simulink model "AirplaneSimModel"  (R2023b)
settings: Solver=ode45  StartTime=0.0  StopTime=inf  RelTol=1e-3
undefined symbols (not defined in the file): aileron_left, aileron_right, airplane, alt_ground, atmosphere, elevator, envir, g, htp_trim, rudder, throttle, wind
libraries: unit_conversions_lib x6, flightgear_visualization_lib x2, joystick_lib x1, conventional_airplane_single_engine_lib x1, atmosphere_lib x1, simulink x1
settings Model: Creator=Yannic  LastModifiedBy=yannic
settings SolverCC: AlgebraicLoopSolver=TrustRegion
settings DataIOCC: ReturnWorkspaceOutputs=off
settings DebuggingCC: UnconnectedInputMsg=warning  UnconnectedOutputMsg=warning  UnconnectedLineMsg=warning  ArithmeticOperatorsInVariantConditions=warning
settings ModelReferenceCC: EnableRefExpFcnMdlSchedulingChecks=on
settings SFSimCC: CustomCodeUndefinedFunction=UseInterfaceOnly

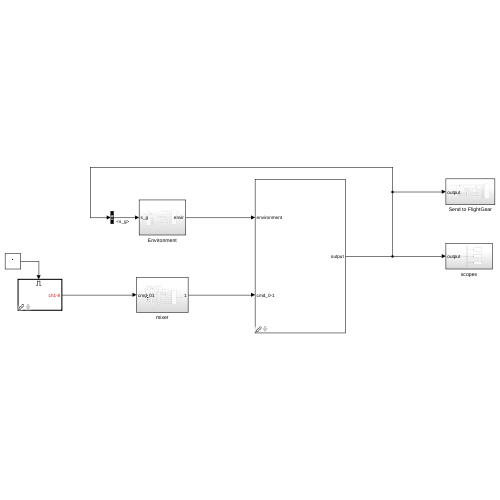
[thumbnail: Simulink's stored preview of the top-level diagram]
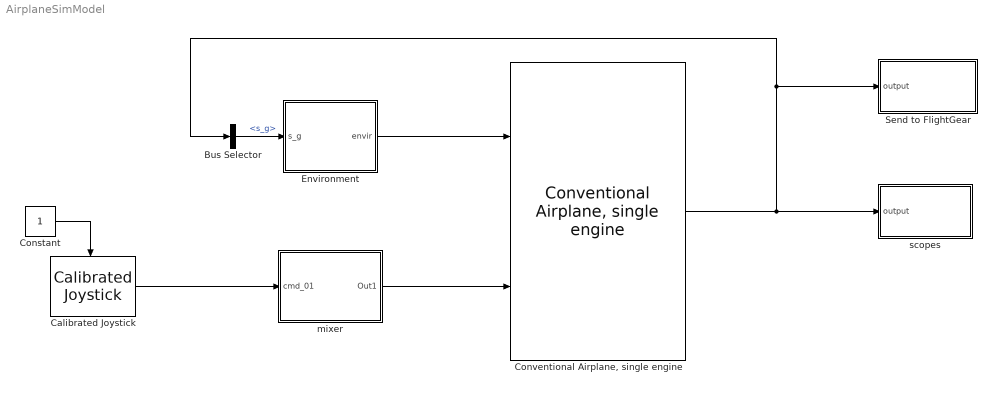
== system AirplaneSimModel ==
  Bus Selector : BusSelector  OutputSignals=rigidBodyBus.s_g
  Calibrated Joystick : joystick_lib/Calibrated Joystick  jystck=jystck  joyid=1
      settings: SourceProductName=LADAC
  Constant : Constant
  "Conventional Airplane, single engine" : conventional_airplane_single_engine_lib/Conventional Airplane, single engine  airplane=airplane
      settings: SourceProductName=LADAC
  Environment : Subsystem
  Send to FlightGear : Subsystem
  mixer : Subsystem
  scopes : Subsystem
  wires:
  Environment/1(envir) -> "Conventional Airplane, single engine"/1
  "Conventional Airplane, single engine"/1 -> Bus Selector/1, Send to FlightGear/1(output), scopes/1(output)
  mixer/1(Out1) -> "Conventional Airplane, single engine"/2
  Bus Selector/1 -> Environment/1(s_g)  "<s_g>"
  Constant/1 -> Calibrated Joystick/Enable
  Calibrated Joystick/1 -> mixer/1(cmd_01)

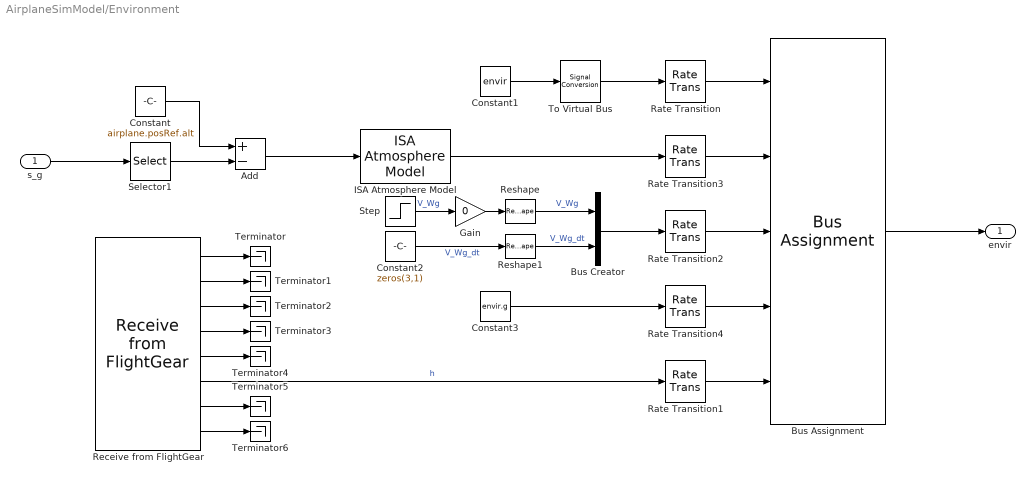
== system AirplaneSimModel/Environment ==
  s_g : Inport
  Add : Sum  Inputs=+-
  Bus Assignment : BusAssignment  AssignedSignals=atmosphere,wind,g,alt_ground
  Bus Creator : BusCreator  Inputs=2
  Constant : Constant  Value=airplane.posRef.alt
  Constant1 : Constant  Value=envir  OutDataTypeStr=Bus: envirBus
  Constant2 : Constant  Value=zeros(3,1)
  Constant3 : Constant  Value=envir.g
  Gain : Gain  Gain=0
  ISA Atmosphere Model : atmosphere_lib/ISA Atmosphere Model
      settings: SourceProductName=LADAC
  Rate Transition{,1..4} (5 alike) : RateTransition
  Receive from FlightGear : flightgear_visualization_lib/Receive from FlightGear  ip_address='127.0.0.1'  ip_port=5503  sample_time=1/40  blocking_time=0  is_aerocntrl=off  is_engine=off  is_fuel=off  is_land=off  is_avionics=off  is_envir=on
      settings: SourceProductName=LADAC
  Reshape : Reshape  OutputDimensionality=Column vector (2-D)
  Reshape1 : Reshape  OutputDimensionality=Column vector (2-D)
  Selector1 : Selector  InputPortWidth=3  IndexOptions=Index vector (dialog)  Indices=3  OutputSizes=1
  Step : Step  Time=3  After=[0;10;0]  SampleTime=0
  Terminator{,1..6} (7 alike) : Terminator
  To Virtual Bus : SignalConversion  ConversionOutput=Virtual bus  OverrideOpt=off
  envir : Outport  VectorParamsAs1DForOutWhenUnconnected=off
  wires:
  Receive from FlightGear/6 -> Rate Transition1/1  "h"
  Rate Transition2/1 -> Bus Assignment/3
  Rate Transition3/1 -> Bus Assignment/2
  Bus Assignment/1 -> envir/1
  Rate Transition/1 -> Bus Assignment/1
  ISA Atmosphere Model/1 -> Rate Transition3/1
  Step/1 -> Gain/1  "V_Wg"
  Rate Transition1/1 -> Bus Assignment/5
  Constant1/1 -> To Virtual Bus/1
  s_g/1 -> Selector1/1
  Bus Creator/1 -> Rate Transition2/1
  Constant2/1 -> Reshape1/1  "V_Wg_dt"
  Rate Transition4/1 -> Bus Assignment/4
  Constant3/1 -> Rate Transition4/1
  Gain/1 -> Reshape/1
  Constant/1 -> Add/1
  Add/1 -> ISA Atmosphere Model/1
  Selector1/1 -> Add/2
  To Virtual Bus/1 -> Rate Transition/1
  Reshape/1 -> Bus Creator/1  "V_Wg"
  Reshape1/1 -> Bus Creator/2  "V_Wg_dt"
  Receive from FlightGear/3 -> Terminator2/1
  Receive from FlightGear/5 -> Terminator4/1
  Receive from FlightGear/1 -> Terminator/1
  Receive from FlightGear/7 -> Terminator5/1
  Receive from FlightGear/2 -> Terminator1/1
  Receive from FlightGear/4 -> Terminator3/1
  Receive from FlightGear/8 -> Terminator6/1

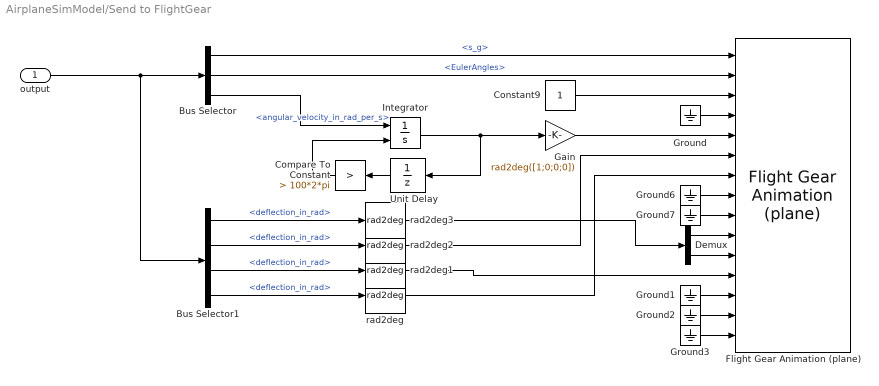
== system AirplaneSimModel/Send to FlightGear ==
  output : Inport
  Bus Selector : BusSelector  OutputSignals=rigidBodyBus.s_g,rigidBodyBus.EulerAngles,actuatorBus.motorBus.angular_velocity_in_rad_per_s
  Bus Selector1 : BusSelector  OutputSignals=actuatorBus.aileronsBus.deflection_in_rad,actuatorBus.elevatorBus.deflection_in_rad,actuatorBus.rudderBus.deflection_in_rad,actuatorBus.htpTrimBus.deflection_in_rad
  Compare To Constant : simulink/Logic and Bit Operations/Compare To Constant  relop=>  const=100*2*pi  OutDataTypeStr=boolean
  Constant9 : Constant
  Demux : Demux  Outputs=2
  Flight Gear Animation (plane) : flightgear_visualization_lib/Flight Gear Animation (plane)  inital_lat=airplane.posRef.lat  inital_long=airplane.posRef.lon  inital_height=airplane.posRef.alt  remoteURL='127.0.0.1'  remotePort=5502
      settings: SourceProductName=LADAC
  Gain : Gain  Gain=rad2deg([1;0;0;0])
  Ground{,1..3,6..7} (6 alike) : Ground
  Integrator : Integrator  ExternalReset=rising
  Unit Delay : UnitDelay  SampleTime=-1  HasFrameUpgradeWarning=on
  rad2deg{,1..3} (4 alike) : unit_conversions_lib/rad2deg
      settings: SourceProductName=LADAC
  wires:
  Compare To Constant/1 -> Integrator/2
  Integrator/1 -> Unit Delay/1, Gain/1
  Bus Selector/1 -> Flight Gear Animation (plane)/1  "<s_g>"
  Bus Selector/2 -> Flight Gear Animation (plane)/2  "<EulerAngles>"
  Gain/1 -> Flight Gear Animation (plane)/5
  Constant9/1 -> Flight Gear Animation (plane)/3
  Unit Delay/1 -> Compare To Constant/1
  Ground/1 -> Flight Gear Animation (plane)/4
  Ground1/1 -> Flight Gear Animation (plane)/13
  Ground2/1 -> Flight Gear Animation (plane)/14
  Ground3/1 -> Flight Gear Animation (plane)/15
  output/1 -> Bus Selector1/1, Bus Selector/1
  Bus Selector/3 -> Integrator/1  "<angular_velocity_in_rad_per_s>"
  Bus Selector1/2 -> rad2deg2/1  "<deflection_in_rad>"
  Bus Selector1/4 -> rad2deg/1  "<deflection_in_rad>"
  Ground6/1 -> Flight Gear Animation (plane)/8
  Ground7/1 -> Flight Gear Animation (plane)/9
  Bus Selector1/3 -> rad2deg1/1  "<deflection_in_rad>"
  Bus Selector1/1 -> rad2deg3/1  "<deflection_in_rad>"
  Demux/1 -> Flight Gear Animation (plane)/10
  Demux/2 -> Flight Gear Animation (plane)/11
  rad2deg/1 -> Flight Gear Animation (plane)/7
  rad2deg1/1 -> Flight Gear Animation (plane)/12
  rad2deg2/1 -> Flight Gear Animation (plane)/6
  rad2deg3/1 -> Demux/1

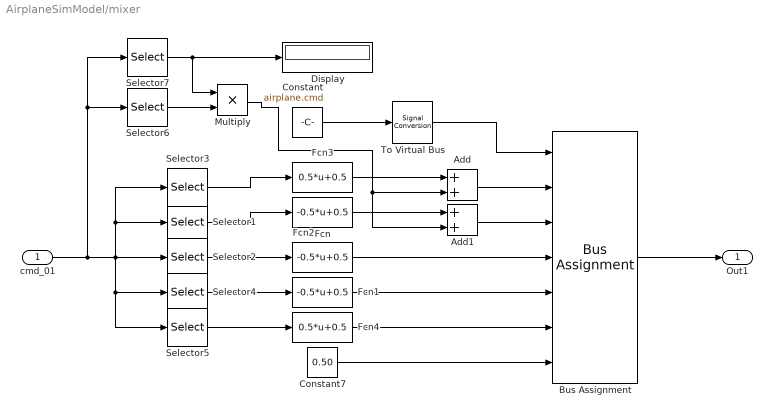
== system AirplaneSimModel/mixer ==
  cmd_01 : Inport
  Add : Sum
  Add1 : Sum
  Bus Assignment : BusAssignment  AssignedSignals=aileron_left,aileron_right,elevator,rudder,throttle,htp_trim
  Constant : Constant  Value=airplane.cmd  OutDataTypeStr=Bus: cmdBus
  Constant7 : Constant  Value=0.50
  Display : Display
  Fcn : Fcn  Expr=-0.5*u+0.5
  Fcn1 : Fcn  Expr=-0.5*u+0.5
  Fcn2 : Fcn  Expr=-0.5*u+0.5
  Fcn3 : Fcn  Expr=0.5*u+0.5
  Fcn4 : Fcn  Expr=0.5*u+0.5
  Multiply : Product
  Selector1 : Selector  InputPortWidth=8  IndexOptions=Index vector (dialog)  Indices=1  OutputSizes=1
  Selector2 : Selector  InputPortWidth=8  IndexOptions=Index vector (dialog)  Indices=2  OutputSizes=1
  Selector3 : Selector  InputPortWidth=8  IndexOptions=Index vector (dialog)  Indices=1  OutputSizes=1
  Selector4 : Selector  InputPortWidth=8  IndexOptions=Index vector (dialog)  Indices=3  OutputSizes=1
  Selector5 : Selector  InputPortWidth=8  IndexOptions=Index vector (dialog)  Indices=4  OutputSizes=1
  Selector6 : Selector  InputPortWidth=8  IndexOptions=Index vector (dialog)  Indices=2  OutputSizes=1
  Selector7 : Selector  InputPortWidth=8  IndexOptions=Index vector (dialog)  Indices=5  OutputSizes=1
  To Virtual Bus : SignalConversion  ConversionOutput=Virtual bus  OverrideOpt=off
  Out1 : Outport  VectorParamsAs1DForOutWhenUnconnected=off
  wires:
  Constant/1 -> To Virtual Bus/1
  Bus Assignment/1 -> Out1/1
  cmd_01/1 -> Selector7/1, Selector6/1, Selector2/1, Selector5/1, Selector4/1, Selector1/1, Selector3/1
  Selector4/1 -> Fcn1/1
  Selector2/1 -> Fcn2/1
  Selector1/1 -> Fcn/1
  Selector3/1 -> Fcn3/1
  Selector5/1 -> Fcn4/1
  Constant7/1 -> Bus Assignment/7
  Fcn1/1 -> Bus Assignment/5
  To Virtual Bus/1 -> Bus Assignment/1
  Fcn2/1 -> Bus Assignment/4
  Fcn4/1 -> Bus Assignment/6
  Selector6/1 -> Multiply/2
  Add/1 -> Bus Assignment/2
  Add1/1 -> Bus Assignment/3
  Fcn3/1 -> Add/1
  Fcn/1 -> Add1/1
  Multiply/1 -> Add1/2, Add/2
  Selector7/1 -> Display/1, Multiply/1

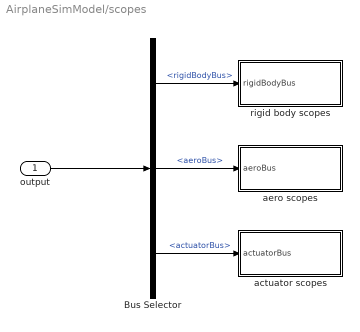
== system AirplaneSimModel/scopes ==
  output : Inport
  Bus Selector : BusSelector  OutputSignals=rigidBodyBus,aeroBus,actuatorBus
  actuator scopes : Subsystem
  aero scopes : Subsystem
  rigid body scopes : Subsystem
  wires:
  Bus Selector/1 -> rigid body scopes/1(rigidBodyBus)  "<rigidBodyBus>"
  Bus Selector/2 -> aero scopes/1(aeroBus)  "<aeroBus>"
  output/1 -> Bus Selector/1
  Bus Selector/3 -> actuator scopes/1(actuatorBus)  "<actuatorBus>"

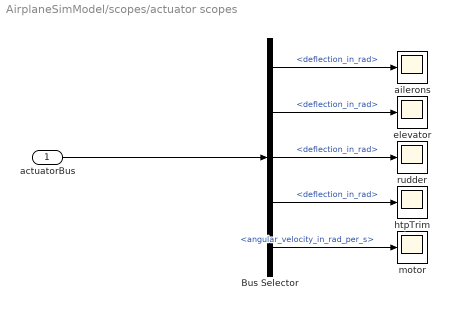
== system AirplaneSimModel/scopes/actuator scopes ==
  actuatorBus : Inport
  Bus Selector : BusSelector  OutputSignals=aileronsBus.deflection_in_rad,elevatorBus.deflection_in_rad,rudderBus.deflection_in_rad,htpTrimBus.deflection_in_rad,motorBus.angular_velocity_in_rad_per_s
  ailerons : Scope
  elevator : Scope
  htpTrim : Scope
  motor : Scope
  rudder : Scope
  wires:
  actuatorBus/1 -> Bus Selector/1
  Bus Selector/1 -> ailerons/1  "<deflection_in_rad>"
  Bus Selector/2 -> elevator/1  "<deflection_in_rad>"
  Bus Selector/3 -> rudder/1  "<deflection_in_rad>"
  Bus Selector/4 -> htpTrim/1  "<deflection_in_rad>"
  Bus Selector/5 -> motor/1  "<angular_velocity_in_rad_per_s>"

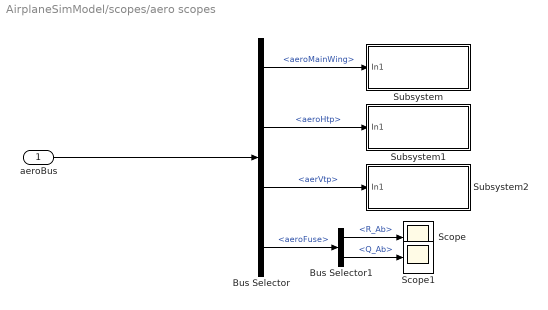
== system AirplaneSimModel/scopes/aero scopes ==
  aeroBus : Inport
  Bus Selector : BusSelector  OutputSignals=aeroMainWing,aeroHtp,aerVtp,aeroFuse
  Bus Selector1 : BusSelector  OutputSignals=R_Ab,Q_Ab
  Scope : Scope
  Scope1 : Scope
  Subsystem : Subsystem
  Subsystem1 : Subsystem
  Subsystem2 : Subsystem
  wires:
  aeroBus/1 -> Bus Selector/1
  Bus Selector/1 -> Subsystem/1(In1)  "<aeroMainWing>"
  Bus Selector/2 -> Subsystem1/1(In1)  "<aeroHtp>"
  Bus Selector/3 -> Subsystem2/1(In1)  "<aerVtp>"
  Bus Selector/4 -> Bus Selector1/1  "<aeroFuse>"
  Bus Selector1/1 -> Scope/1  "<R_Ab>"
  Bus Selector1/2 -> Scope1/1  "<Q_Ab>"

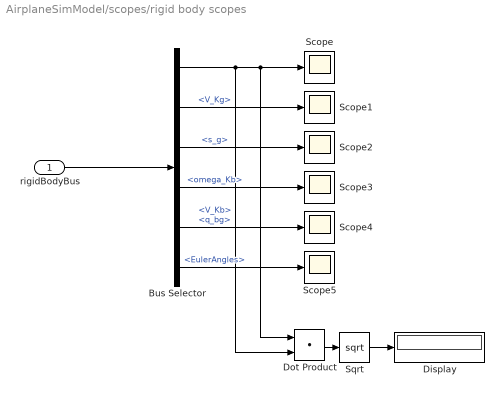
== system AirplaneSimModel/scopes/rigid body scopes ==
  rigidBodyBus : Inport
  Bus Selector : BusSelector  OutputSignals=V_Kb,V_Kg,s_g,omega_Kb,q_bg,EulerAngles
  Display : Display
  Dot Product : DotProduct  OutDataTypeStr=Inherit: Inherit via internal rule
  Scope{,1..5} (6 alike) : Scope
  Sqrt : Sqrt
  wires:
  rigidBodyBus/1 -> Bus Selector/1
  Bus Selector/1 -> Dot Product/2, Dot Product/1, Scope/1  "<V_Kb>"
  Bus Selector/2 -> Scope1/1  "<V_Kg>"
  Bus Selector/3 -> Scope2/1  "<s_g>"
  Bus Selector/4 -> Scope3/1  "<omega_Kb>"
  Bus Selector/5 -> Scope4/1  "<q_bg>"
  Bus Selector/6 -> Scope5/1  "<EulerAngles>"
  Dot Product/1 -> Sqrt/1
  Sqrt/1 -> Display/1

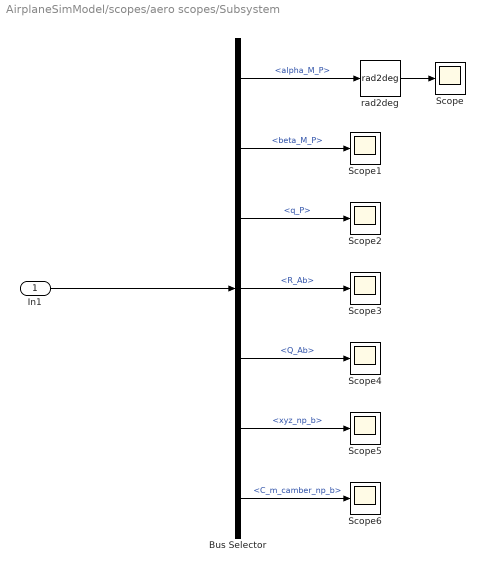
== system AirplaneSimModel/scopes/aero scopes/Subsystem ==
  In1 : Inport
  Bus Selector : BusSelector  OutputSignals=aeroAxes.alpha_M_P,aeroAxes.beta_M_P,aeroAxes.q_P,dynamicsBody.R_Ab,dynamicsBody.Q_Ab,dynamicsBody.xyz_np_b,dynamicsBody.C_m_camber_np_b
  Scope{,1..6} (7 alike) : Scope
  rad2deg : unit_conversions_lib/rad2deg
      settings: SourceProductName=LADAC
  wires:
  In1/1 -> Bus Selector/1
  Bus Selector/1 -> rad2deg/1  "<alpha_M_P>"
  Bus Selector/3 -> Scope2/1  "<q_P>"
  Bus Selector/2 -> Scope1/1  "<beta_M_P>"
  Bus Selector/4 -> Scope3/1  "<R_Ab>"
  Bus Selector/5 -> Scope4/1  "<Q_Ab>"
  Bus Selector/6 -> Scope5/1  "<xyz_np_b>"
  Bus Selector/7 -> Scope6/1  "<C_m_camber_np_b>"
  rad2deg/1 -> Scope/1

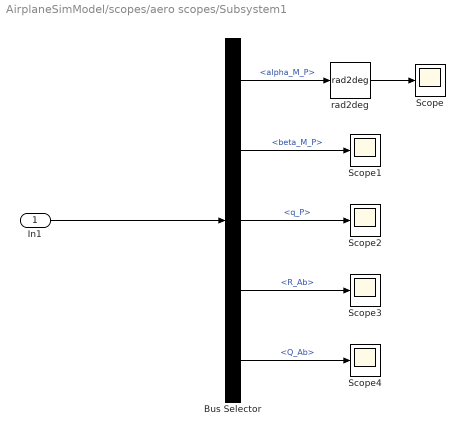
== system AirplaneSimModel/scopes/aero scopes/Subsystem1 ==
  In1 : Inport
  Bus Selector : BusSelector  OutputSignals=aeroAxes.alpha_M_P,aeroAxes.beta_M_P,aeroAxes.q_P,dynamicsBody.R_Ab,dynamicsBody.Q_Ab
  Scope{,1..4} (5 alike) : Scope
  rad2deg : unit_conversions_lib/rad2deg
      settings: SourceProductName=LADAC
  wires:
  Bus Selector/5 -> Scope4/1  "<Q_Ab>"
  Bus Selector/4 -> Scope3/1  "<R_Ab>"
  Bus Selector/2 -> Scope1/1  "<beta_M_P>"
  Bus Selector/3 -> Scope2/1  "<q_P>"
  Bus Selector/1 -> rad2deg/1  "<alpha_M_P>"
  In1/1 -> Bus Selector/1
  rad2deg/1 -> Scope/1

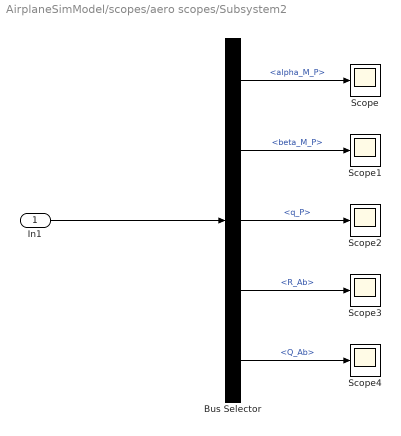
== system AirplaneSimModel/scopes/aero scopes/Subsystem2 ==
  In1 : Inport
  Bus Selector : BusSelector  OutputSignals=aeroAxes.alpha_M_P,aeroAxes.beta_M_P,aeroAxes.q_P,dynamicsBody.R_Ab,dynamicsBody.Q_Ab
  Scope{,1..4} (5 alike) : Scope
  wires:
  In1/1 -> Bus Selector/1
  Bus Selector/1 -> Scope/1  "<alpha_M_P>"
  Bus Selector/3 -> Scope2/1  "<q_P>"
  Bus Selector/2 -> Scope1/1  "<beta_M_P>"
  Bus Selector/4 -> Scope3/1  "<R_Ab>"
  Bus Selector/5 -> Scope4/1  "<Q_Ab>"
